simulink model "labaZB2"  (R2022a)
settings: Solver=VariableStepAuto  StartTime=0.0  StopTime=10  RelTol=1e-3
settings Model: Creator=User  LastModifiedBy=salgi

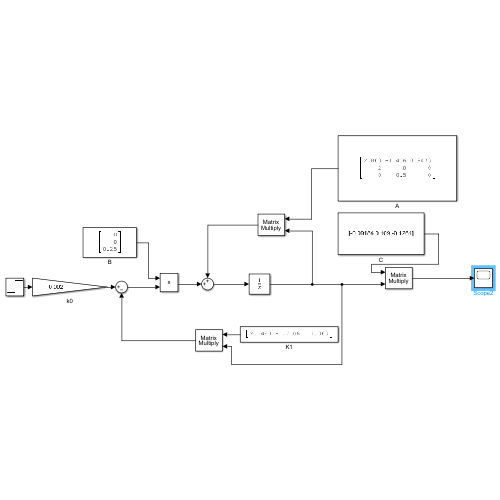
[thumbnail: Simulink's stored preview of the top-level diagram]
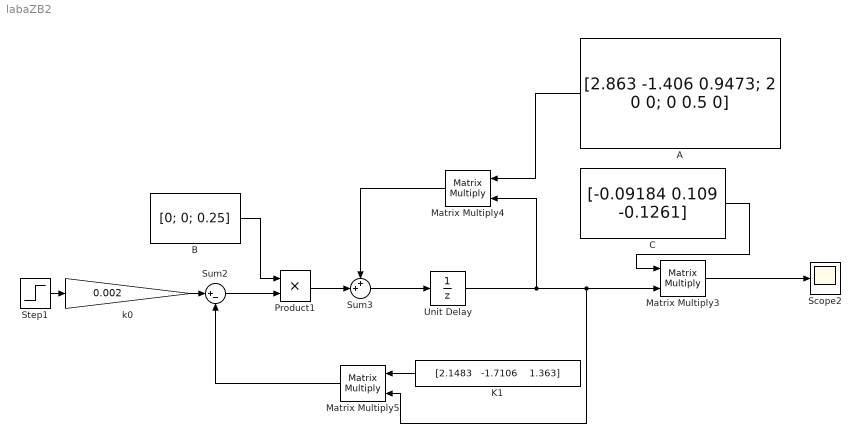
== system labaZB2 ==
  A : Constant  Value="[2.863  -1.406  0.9473; 2 0 0; 0 0.5 0]"  VectorParams1D=off
  B : Constant  Value=[0; 0; 0.25]  VectorParams1D=off
  C : Constant  Value=[-0.09184 0.109 -0.1261]  VectorParams1D=off
  K1 : Constant  Value="[2.1483   -1.7106    1.363]"  VectorParams1D=off
  Matrix Multiply3 : Product  Multiplication=Matrix(*)
  Matrix Multiply4 : Product  Multiplication=Matrix(*)
  Matrix Multiply5 : Product  Multiplication=Matrix(*)
  Product1 : Product
  Scope2 : Scope
  Step1 : Step  Time=0  SampleTime=10
  Sum2 : Sum  Inputs=|+-
  Sum3 : Sum  Inputs=++|
  Unit Delay : UnitDelay  SampleTime=10  HasFrameUpgradeWarning=on
  k0 : Gain  Gain=0.002
  wires:
  Matrix Multiply3/1 -> Scope2/1
  Sum3/1 -> Unit Delay/1
  B/1 -> Product1/1
  Step1/1 -> k0/1
  Unit Delay/1 -> Matrix Multiply5/2, Matrix Multiply3/2, Matrix Multiply4/2
  Product1/1 -> Sum3/2
  k0/1 -> Sum2/1
  Sum2/1 -> Product1/2
  Matrix Multiply5/1 -> Sum2/2
  Matrix Multiply4/1 -> Sum3/1
  C/1 -> Matrix Multiply3/1
  A/1 -> Matrix Multiply4/1
  K1/1 -> Matrix Multiply5/1
